simulink model "ark_io_codegen_check"  (R2024b)
settings: Solver=FixedStepDiscrete  StartTime=0.0  StopTime=0.005  FixedStep=0.001  RelTol=1e-3
libraries: x280_dio_library x4, x280_serial_library x3
settings Model: Creator=yonggang.zhang  LastModifiedBy=yonggang.zhang
settings OptimizationCC: EnhancedBackFolding=on  PassReuseOutputArgsAs=Individual arguments  ZeroExternalMemoryAtStartup=off  ZeroInternalMemoryAtStartup=off  MaxStackSize=64  OptimizeBlockOrder=speed  DifferentSizesBufferReuse=on  OptimizationCustomize=off  EfficientTunableParamExpr=on
settings DebuggingCC: ParameterTunabilityLossMsg=error
settings HardwareCC: ProdBitPerLong=64  ProdHWDeviceType=Intel->x86-64 (Linux 64)
settings SFSimCC: MATLABDynamicMemAlloc=off
settings RTWCC: Description=Embedded Coder  SystemTargetFile=ert.tlc  HardwareBoard=SimRT  TLCOptions="-aInlineSetEventsForThisBaseRateFcn=TLC_FALSE -aSuppressMultiTaskScheduler=TLC_FALSE  -aRateBasedStepFcn=0"  TemplateMakefile=ert_default_tmf  Toolchain=X280 portable-linux-toolchain
settings CodeAppCC: ForceParamTrailComments=on  IgnoreCustomStorageClasses=off  OperatorAnnotations=on  SimulinkDataObjDesc=on  SFDataObjDesc=on  InsertBlockDesc=on
settings ERTTargetCC: ExtMode=on  ExtModeTransport=2  ExtModeStaticAlloc=on  ExtModeMexFile=ext_xcp  ExtModeIntrfLevel=Level2 - Open  InlinedParameterPlacement=Hierarchical

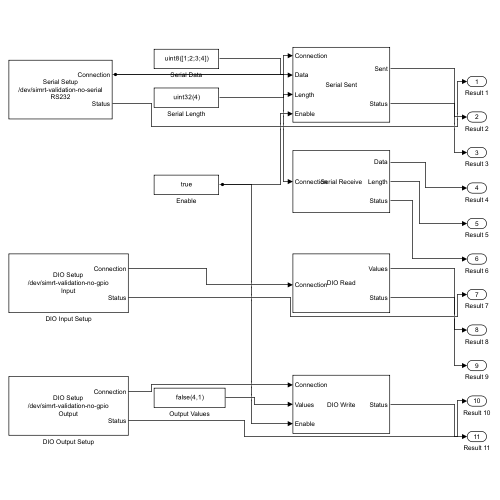
[thumbnail: Simulink's stored preview of the top-level diagram]
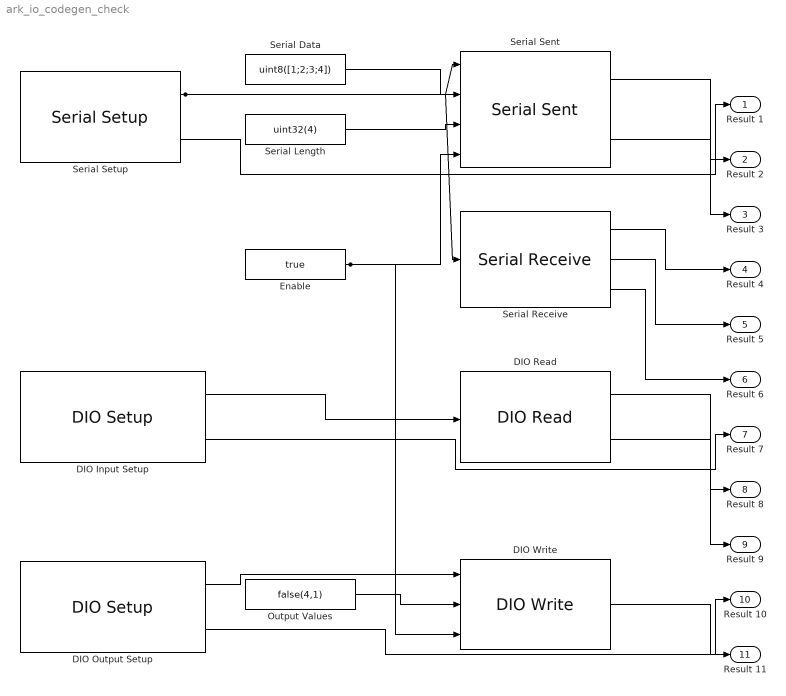
== system ark_io_codegen_check ==
  DIO Input Setup : x280_dio_library/DIO Setup  Device=/dev/simrt-validation-no-gpio  LineOffsets=[0 1 2 3]  Direction=Input  ActiveLow=false  InitialValues=false  SampleTime=0.001
      settings: SourceProductName=X280 Linux Digital IO
  DIO Output Setup : x280_dio_library/DIO Setup  Device=/dev/simrt-validation-no-gpio  LineOffsets=[4 5 6 7]  Direction=Output  ActiveLow=false  InitialValues=false  SampleTime=0.001
      settings: SourceProductName=X280 Linux Digital IO
  DIO Read : x280_dio_library/DIO Read  LineCount=4
      settings: SourceProductName=X280 Linux Digital IO
  DIO Write : x280_dio_library/DIO Write
      settings: SourceProductName=X280 Linux Digital IO
  Enable : Constant  Value=true  SampleTime=0.001
  Output Values : Constant  Value=false(4,1)  SampleTime=0.001
  Serial Data : Constant  Value=uint8([1;2;3;4])  SampleTime=0.001
  Serial Length : Constant  Value=uint32(4)  SampleTime=0.001
  Serial Receive : x280_serial_library/Serial Receive  BufferSize=16
      settings: SourceProductName=X280 Linux Serial
  Serial Sent : x280_serial_library/Serial Sent
      settings: SourceProductName=X280 Linux Serial
  Serial Setup : x280_serial_library/Serial Setup  Device=/dev/simrt-validation-no-serial  BaudRate=115200  DataBits=8  Parity=None  StopBits=1  Mode=RS232  RS485Direction=Hardware auto  RTSOnSend=true  DelayBeforeSendMs=0  DelayAfterSendMs=0  SampleTime=0.001
      settings: SourceProductName=X280 Linux Serial
  Result 1 : Outport
  Result 2 : Outport  Port=2
  Result 3 : Outport  Port=3
  Result 4 : Outport  Port=4
  Result 5 : Outport  Port=5
  Result 6 : Outport  Port=6
  Result 7 : Outport  Port=7
  Result 8 : Outport  Port=8
  Result 9 : Outport  Port=9
  Result 10 : Outport  Port=10
  Result 11 : Outport  Port=11
  wires:
  Serial Setup/1 -> Serial Sent/1, Serial Receive/1
  Serial Data/1 -> Serial Sent/2
  Serial Length/1 -> Serial Sent/3
  Enable/1 -> Serial Sent/4, DIO Write/3
  DIO Input Setup/1 -> DIO Read/1
  DIO Output Setup/1 -> DIO Write/1
  Output Values/1 -> DIO Write/2
  Serial Setup/2 -> Result 1/1
  Serial Sent/1 -> Result 2/1
  Serial Sent/2 -> Result 3/1
  Serial Receive/1 -> Result 4/1
  Serial Receive/2 -> Result 5/1
  Serial Receive/3 -> Result 6/1
  DIO Input Setup/2 -> Result 7/1
  DIO Read/1 -> Result 8/1
  DIO Read/2 -> Result 9/1
  DIO Output Setup/2 -> Result 10/1
  DIO Write/1 -> Result 11/1
